simulink model "QDrone_YOLO_Integrated_Camera_Commander"  (R2021b)
settings: Solver=ode1  StartTime=0.0  StopTime=inf  FixedStep=0.001  RelTol=1e-3  EnableMultiTasking=on
InitFcn:
  | set_param(gcs, 'ZoomFactor','FitSystem')
model workspace (MAT data in the model file):
  target_system = 1
undefined symbols (not defined in the file): gcbh, HIL, JPEG, qc_get_step_size, video_display_show
libraries: quarc_library x53, simulink x23, simulink_extras x5
(part 2 of 3)

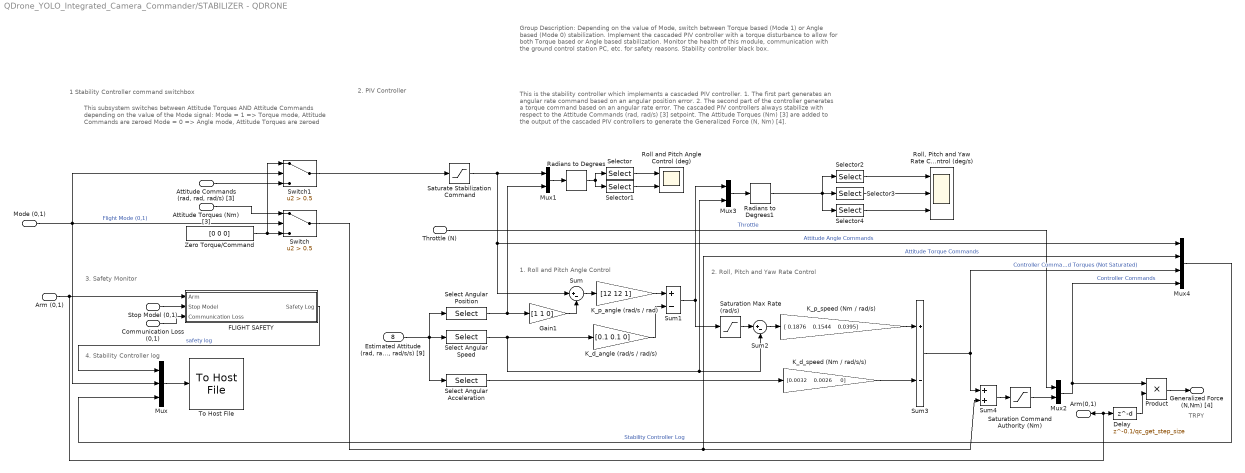
== system QDrone_YOLO_Integrated_Camera_Commander/STABILIZER - QDRONE  ==
  note: 2. PIV Controller
  note: 4. Stability Controller log
  note: 1 Stability Controller command switchbox
  note: Group Description:
      |
      | Depending on the value of Mode, switch between Torque based (Mode 1) or Angle based (Mode 0) stabilization.
      | Implement the cascaded PIV controller with a torque disturbance to allow for both Torque based or Angle based stabilization.
      | Monitor the health of this module, communication with the ground control station PC, etc. for safety reasons.
      | Stability controller black box.
  note: TRPY
  note: 2. Roll, Pitch and Yaw Rate Control
  note: 1. Roll and Pitch Angle Control
  note: This is the stability controller which implements a cascaded PIV controller.
      | 1. The first part generates an angular rate command based on an angular position error.
      | 2. The second part of the controller generates a torque command based on an angular rate error.
      |
      | The cascaded PIV controllers always stabilize with respect to the Attitude Commands (rad, rad/s) [3] setpoint. The Attitude Torques (Nm) [3] are added to the output of the cascaded PIV controllers to generate the Generalized Force (N, Nm) [4].
  note: This subsystem switches between Attitude Torques AND Attitude Commands depending on
      | the value of the Mode signal:
      | Mode = 1	=> 		Torque mode, Attitude Commands are zeroed
      | Mode = 0	=> 		Angle mode, Attitude Torques are zeroed
  note: 3. Safety Monitor
  Mode (0,1) : Inport
  Stop Model (0,1) : Inport  Port=2
  Throttle (N) : Inport  Port=3
  Attitude Torques (Nm) [3] : Inport  Port=4
  "Attitude Commands (rad, rad, rad/s) [3]" : Inport  Port=5
  Communication Loss (0,1) : Inport  Port=6
  Arm (0,1) : Inport  Port=7
  "Estimated Attitude (rad, rad/s, rad/s/s) [9]" : Inport  Port=8
  Delay : Delay  DelayLength=0.1/qc_get_step_size
  FLIGHT SAFETY : Subsystem
  Gain1 : Gain  Gain=[1 1 0]
  K_d_angle (rad/s / rad/s) : Gain  Gain=[0.1 0.1 0]
  K_d_speed (Nm / rad/s/s) : Gain  Gain="[0.0032    0.0026     0]"
  K_p_angle (rad/s / rad) : Gain  Gain=[12 12 1]
  K_p_speed (Nm / rad/s) : Gain  Gain="[ 0.1876    0.1544    0.0395]"
  Mux : Mux  Inputs=3
  Mux1 : Mux  Inputs=2
  Mux2 : Mux  Inputs=2
  Mux3 : Mux  Inputs=2
  Mux4 : Mux
  Product : Product
  Radians to Degrees : simulink_extras/Transformations/Radians to Degrees
  Radians to Degrees1 : simulink_extras/Transformations/Radians to Degrees
  Roll and Pitch Angle Control (deg) : Scope  NumInputPorts=2
  "Roll, Pitch and Yaw Rate Control (deg/s)" : Scope  NumInputPorts=3
  Saturate Stabilization Command : Saturate  UpperLimit=[pi/4 pi/4 10*pi/18]  LowerLimit=[-pi/4 -pi/4 -10*pi/18]
  Saturation Command Authority (Nm) : Saturate  UpperLimit=[1.0915 0.8984 0.0984]  LowerLimit=-[1.0915 0.8984 0.0984]
  Saturation Max Rate (rad/s) : Saturate  UpperLimit=10*pi/3*[1 1 1]  LowerLimit=-10*pi/3*[1 1 1]
  Select Angular Acceleration : Selector  InputPortWidth=9  IndexOptions=Index vector (dialog)  Indices=[7:9]  OutputSizes=1
  Select Angular Speed : Selector  InputPortWidth=9  IndexOptions=Index vector (dialog)  Indices=[4:6]  OutputSizes=1
  Select Angular Position : Selector  InputPortWidth=9  IndexOptions=Index vector (dialog)  Indices=[1:3]  OutputSizes=1
  Selector : Selector  InputPortWidth=6  IndexOptions=Index vector (dialog)  Indices=[1 4]  OutputSizes=1
  Selector1 : Selector  InputPortWidth=6  IndexOptions=Index vector (dialog)  Indices=[2 5]  OutputSizes=1
  Selector2 : Selector  InputPortWidth=6  IndexOptions=Index vector (dialog)  Indices=[1 4]  OutputSizes=1
  Selector3 : Selector  InputPortWidth=6  IndexOptions=Index vector (dialog)  Indices=[2 5]  OutputSizes=1
  Selector4 : Selector  InputPortWidth=6  IndexOptions=Index vector (dialog)  Indices=[3 6]  OutputSizes=1
  Sum : Sum  Inputs=|+-
  Sum1 : Sum  Inputs=+-
  Sum2 : Sum  Inputs=|+-
  Sum3 : Sum  Inputs=+-
  Sum4 : Sum
  Switch : Switch  Criteria=u2 > Threshold  Threshold=0.5
  Switch1 : Switch  Criteria=u2 > Threshold  Threshold=0.5
  To Host File : quarc_library/Sinks/To Host/To Host File  file_name=saved_data/%m/Stabilizer_%{date}_%{time}.mat  variable_name=stabilizer_data  decimation=1  sample_time=-1  file_format=MAT-file v.5  options=No header or footer  append=off  final_file_name=saved_data/QDrone_YOLO_Integrated_Camera_Commander/Stabilizer_19-Aug-2026_13-55-19.mat  bitrate=2000000
      settings: SourceProductName=The database C:\Users\user\AppData\Roaming\MathWorks\MATLAB\R2017a\slblocks_master.db is locked, or a table in the database is locked. (database is locked)
  Zero Torque/Command : Constant  Value=[0 0 0]
  Generalized Force (N,Nm) [4] : Outport  VectorParamsAs1DForOutWhenUnconnected=off
  Arm(0,1) : Outport  Port=2  VectorParamsAs1DForOutWhenUnconnected=off
  wires:
  Product/1 -> Generalized Force (N,Nm) [4]/1
  Stop Model (0,1)/1 -> FLIGHT SAFETY/2(Stop Model)
  Communication Loss (0,1)/1 -> FLIGHT SAFETY/3(Communication Loss)
  Mux/1 -> To Host File/1
  Mux4/1 -> Mux/3  "Stability Controller Log"
  Mode (0,1)/1 -> Switch/2, Switch1/2, Mux/2  "Flight Mode (0,1)"
  FLIGHT SAFETY/1(Safety Log) -> Mux/1  "safety log"
  K_p_speed (Nm / rad/s)/1 -> Sum3/1
  Sum/1 -> K_p_angle (rad/s / rad)/1
  K_d_speed (Nm / rad/s/s)/1 -> Sum3/2
  Arm (0,1)/1 -> Arm(0,1)/1, Delay/1, FLIGHT SAFETY/1(Arm)
  Mux3/1 -> Radians to Degrees1/1
  Sum1/1 -> Saturation Max Rate (rad/s)/1, Mux3/1
  Saturate Stabilization Command/1 -> Mux1/1, Sum/1, Mux4/1  "Attitude Angle Commands"
  Mux2/1 -> Mux4/4, Product/1  "Controller Commands"
  Select Angular Position/1 -> Mux1/2, Gain1/1
  Sum2/1 -> K_p_speed (Nm / rad/s)/1
  Throttle (N)/1 -> Mux2/1  "Throttle"
  Selector1/1 -> Roll and Pitch Angle Control (deg)/2
  Switch/1 -> Mux4/2, Sum4/2  "Attitude Torque Commands"
  Radians to Degrees1/1 -> Selector2/1, Selector4/1, Selector3/1
  "Estimated Attitude (rad, rad/s, rad/s/s) [9]"/1 -> Select Angular Position/1, Select Angular Acceleration/1, Select Angular Speed/1
  Mux1/1 -> Radians to Degrees/1
  Selector3/1 -> "Roll, Pitch and Yaw Rate Control (deg/s)"/2
  Sum4/1 -> Saturation Command Authority (Nm)/1
  Sum3/1 -> Mux4/3, Sum4/1  "Controller Command Torques (Not Saturated)"
  Saturation Command Authority (Nm)/1 -> Mux2/2
  Gain1/1 -> Sum/2
  Select Angular Acceleration/1 -> K_d_speed (Nm / rad/s/s)/1
  Switch1/1 -> Saturate Stabilization Command/1
  Saturation Max Rate (rad/s)/1 -> Sum2/1
  Selector4/1 -> "Roll, Pitch and Yaw Rate Control (deg/s)"/3
  K_p_angle (rad/s / rad)/1 -> Sum1/1
  Select Angular Speed/1 -> Sum2/2, Mux3/2, K_d_angle (rad/s / rad/s)/1
  Selector/1 -> Roll and Pitch Angle Control (deg)/1
  Selector2/1 -> "Roll, Pitch and Yaw Rate Control (deg/s)"/1
  K_d_angle (rad/s / rad/s)/1 -> Sum1/2
  Radians to Degrees/1 -> Selector/1, Selector1/1
  "Attitude Commands (rad, rad, rad/s) [3]"/1 -> Switch1/3
  Attitude Torques (Nm) [3]/1 -> Switch/1
  Zero Torque/Command/1 -> Switch1/1, Switch/3
  Delay/1 -> Product/2

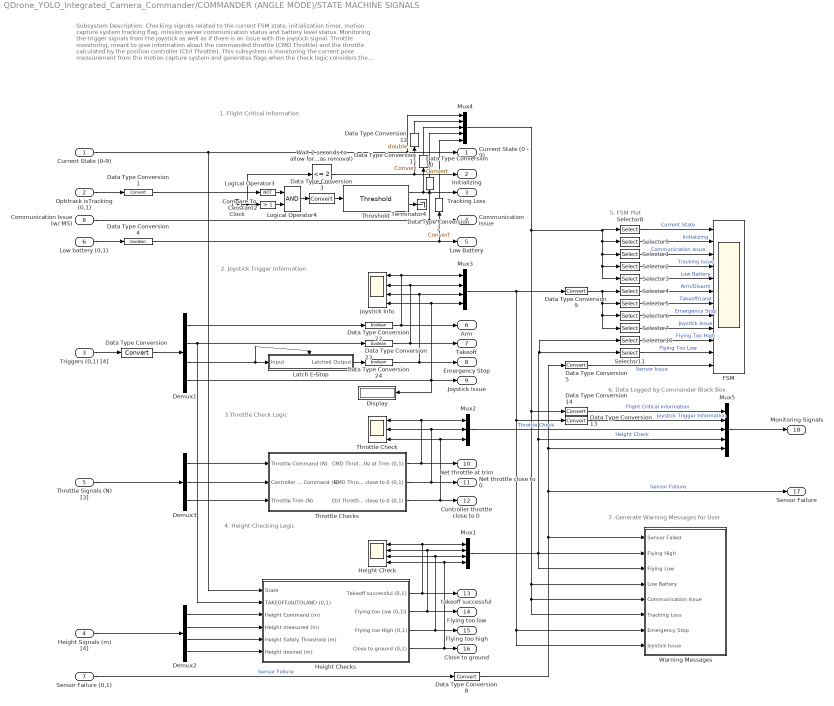
== system QDrone_YOLO_Integrated_Camera_Commander/COMMANDER (ANGLE MODE)/STATE MACHINE SIGNALS ==
  note: Subsystem Description:
      | Checking signals related to the current FSM state, initialization timer, motion capture system tracking flag, mission server communication status and battery level status.
      | Monitoring the trigger signals from the joystick as well as if there is an issue with the joystick signal.
      | Throttle monitoring, meant to give information about the commanded throttle (CMD Throttle) and the throttle calculated by the position controller (Ctrl Throttle).
      | This subsystem is monitoring the current pose measurement from the motion capture system and generates flags when the check logic considers the QDrone flying to close to ground, too high or too low as well as generate a successful take off flag.
      | A subset of the FSM monitoring signals are shown using this scope. These signals are what Quanser considers importnat for flight.
      | FSM signals sent to the blackbox for post flight monitoring.
      | Error message generation based on flags generated by the FSM signal checks.
  note: 7. Generate Warning Messages for User
  note: 5. FSM Plot
  note: 6. Data Logged by Commander Black Box
  note: 1. Flight Critical Information
  note: 2. Joystick Trigger Information
  note: 3.Throttle Check Logic
  note: 4. Height Checking Logic
  Current State (0-9) : Inport
  "Optitrack isTracking (0,1)  " : Inport  Port=2
  Triggers (0,1) [4] : Inport  Port=3
  Height Signals (m) [4] : Inport  Port=4
  Throttle Signals (N) [3] : Inport  Port=5
  Low battery (0,1) : Inport  Port=6
  Sensor Failure (0,1) : Inport  Port=7
  Communication Issue (w/ MS) : Inport  Port=8
  Clock : Clock
  Compare To Constant2 : simulink/Logic and Bit Operations/Compare To Constant  relop=>  const=1  OutDataTypeStr=boolean
  Data Type Conversion{,1..3,5,8..11,13..14} (11 alike) : DataTypeConversion
  Data Type Conversion12 : DataTypeConversion  OutDataTypeStr=double
  Data Type Conversion{4,22..24} (4 alike) : DataTypeConversion  OutDataTypeStr=boolean
  Demux1 : Demux  Outputs=[1 1 1 1]
  Demux2 : Demux
  Demux3 : Demux  Outputs=3
  Display : Display
  FSM : Scope  NumInputPorts=12
  "Height Check " : Scope  NumInputPorts=4
  Height Checks : Subsystem
  Joystick Info : Scope  NumInputPorts=4
  Latch E-Stop : Subsystem  TreatAsAtomicUnit=on
  Logical Operator3 : Logic  Operator=NOT  AllPortsSameDT=off  OutDataTypeStr=boolean
  Logical Operator4 : Logic  AllPortsSameDT=off  OutDataTypeStr=boolean
  Mux1 : Mux  Inputs=[1 1 1 1]
  Mux2 : Mux  Inputs=[1 1 1]
  Mux3 : Mux  Inputs=[1 1 1 1]
  Mux4 : Mux  Inputs=[1 1 1 1 1]
  Mux5 : Mux  Inputs=[5 4 3 4 1]
  Selector1 : Selector  InputPortWidth=5  IndexOptions=Index vector (dialog)  Indices=4  OutputSizes=1
  Selector10 : Selector  InputPortWidth=4  IndexOptions=Index vector (dialog)  Indices=3  OutputSizes=1
  Selector11 : Selector  InputPortWidth=4  IndexOptions=Index vector (dialog)  Indices=2  OutputSizes=1
  Selector2 : Selector  InputPortWidth=5  IndexOptions=Index vector (dialog)  Indices=3  OutputSizes=1
  Selector3 : Selector  InputPortWidth=5  IndexOptions=Index vector (dialog)  Indices=5  OutputSizes=1
  Selector4 : Selector  InputPortWidth=4  IndexOptions=Index vector (dialog)  Indices=1  OutputSizes=1
  Selector5 : Selector  InputPortWidth=4  IndexOptions=Index vector (dialog)  Indices=2  OutputSizes=1
  Selector6 : Selector  InputPortWidth=4  IndexOptions=Index vector (dialog)  Indices=3  OutputSizes=1
  Selector7 : Selector  InputPortWidth=4  IndexOptions=Index vector (dialog)  Indices=4  OutputSizes=1
  Selector8 : Selector  InputPortWidth=5  IndexOptions=Index vector (dialog)  Indices=1  OutputSizes=1
  Selector9 : Selector  InputPortWidth=5  IndexOptions=Index vector (dialog)  Indices=2  OutputSizes=1
  Terminator4 : Terminator
  Threshold : quarc_library/Discontinuities/Threshold  operator=>=  param_src=Specify via dialog  threshold=0.5  duration=0.2
      settings: SourceProductName=QUARC Targets
  Throttle Check : Scope  NumInputPorts=3
  Throttle Checks : Subsystem
  "Wait 2 seconds to allow for initialization (e.g., bias removal)" : simulink/Logic and Bit Operations/Compare To Constant  relop=<=  const=2  OutDataTypeStr=boolean
  Warning Messages : Subsystem
  "Current State (0 - 9)  " : Outport  VectorParamsAs1DForOutWhenUnconnected=off
  Initializing : Outport  Port=2  VectorParamsAs1DForOutWhenUnconnected=off
  Tracking Loss : Outport  Port=3  VectorParamsAs1DForOutWhenUnconnected=off
  Communication Issue : Outport  Port=4  VectorParamsAs1DForOutWhenUnconnected=off
  Low Battery : Outport  Port=5  VectorParamsAs1DForOutWhenUnconnected=off
  Arm : Outport  Port=6  VectorParamsAs1DForOutWhenUnconnected=off
  Takeoff : Outport  Port=7  VectorParamsAs1DForOutWhenUnconnected=off
  Emergency Stop : Outport  Port=8  VectorParamsAs1DForOutWhenUnconnected=off
  "Joystick Issue " : Outport  Port=9  VectorParamsAs1DForOutWhenUnconnected=off
  Net throttle at trim : Outport  Port=10  VectorParamsAs1DForOutWhenUnconnected=off
  Net throttle close to 0 : Outport  Port=11  VectorParamsAs1DForOutWhenUnconnected=off
  Controller throttle close to 0 : Outport  Port=12  VectorParamsAs1DForOutWhenUnconnected=off
  takeoff successful : Outport  Port=13  VectorParamsAs1DForOutWhenUnconnected=off
  Flying too low : Outport  Port=14  VectorParamsAs1DForOutWhenUnconnected=off
  Flying too high : Outport  Port=15  VectorParamsAs1DForOutWhenUnconnected=off
  Close to ground : Outport  Port=16  VectorParamsAs1DForOutWhenUnconnected=off
  "  Sensor Failure" : Outport  Port=17  VectorParamsAs1DForOutWhenUnconnected=off
  Monitoring Signals : Outport  Port=18  VectorParamsAs1DForOutWhenUnconnected=off
  wires:
  Triggers (0,1) [4]/1 -> Data Type Conversion/1
  Demux2/1 -> Height Checks/3(Height Command (m))
  Demux3/1 -> Throttle Checks/1(Throttle Command (N))
  Height Signals (m) [4]/1 -> Demux2/1
  Demux2/4 -> Height Checks/6(Height desired (m))
  Throttle Signals (N) [3]/1 -> Demux3/1
  Demux1/1 -> Data Type Conversion22/1
  Throttle Checks/2(CMD Throttle close to 0 (0,1)) -> Mux2/2, Throttle Check/2, Net throttle close to 0/1
  Height Checks/1(Takeoff successful (0,1)) -> takeoff successful/1, "Height Check "/1, Mux1/1
  Demux2/3 -> Height Checks/5(Height Safety Threshold (m))
  Demux1/2 -> Data Type Conversion23/1, Height Checks/2(TAKEOFF/AUTOLAND (0,1))
  Demux2/2 -> Height Checks/4(Height measured (m))
  Demux3/2 -> Throttle Checks/2(Controller Throttle Command (N))
  Demux3/3 -> Throttle Checks/3(Throttle Trim (N))
  Throttle Checks/1(CMD Throttle at Trim (0,1)) -> Net throttle at trim/1, Mux2/1, Throttle Check/1
  Height Checks/3(Flying too High (0,1)) -> Mux1/3, "Height Check "/3, Flying too high/1
  Height Checks/4(Close to ground (0,1)) -> "Height Check "/4, Mux1/4, Close to ground/1
  Data Type Conversion/1 -> Demux1/1
  Low battery (0,1)/1 -> Data Type Conversion4/1
  Height Checks/2(Flying too Low (0,1l)) -> Flying too low/1, Mux1/2, "Height Check "/2
  Sensor Failure (0,1)/1 -> Data Type Conversion8/1  "Sensor Failure"
  Data Type Conversion1/1 -> Logical Operator3/1
  Data Type Conversion3/1 -> Threshold/1
  Compare To Constant2/1 -> Logical Operator4/2
  Clock/1 -> "Wait 2 seconds to allow for initialization (e.g., bias removal)"/1, Compare To Constant2/1
  Logical Operator4/1 -> Data Type Conversion3/1
  Threshold/2 -> Terminator4/1
  Logical Operator3/1 -> Logical Operator4/1
  "Optitrack isTracking (0,1)  "/1 -> Data Type Conversion1/1
  Latch E-Stop/1(Latched Output) -> Data Type Conversion24/1
  Demux1/3 -> Latch E-Stop/1(Input), Latch E-Stop/Trigger
  Selector9/1 -> FSM/2  "Initializing"
  Selector1/1 -> FSM/3  "Communication Issue"
  Selector2/1 -> FSM/4  "Tracking Issue"
  Selector3/1 -> FSM/5  "Low Battery"
  Selector4/1 -> FSM/6  "Arm/Disarm"
  Selector5/1 -> FSM/7  "Takeoff/Land"
  Selector6/1 -> FSM/8  "Emergency Stop"
  Selector7/1 -> FSM/9  "Joystick Issue"
  Data Type Conversion5/1 -> FSM/12  "Sensor Issue"
  Selector10/1 -> FSM/10  "Flying Too High"
  Selector11/1 -> FSM/11  "Flying Too Low"
  Data Type Conversion24/1 -> Joystick Info/3, Mux3/3, Emergency Stop/1
  Data Type Conversion23/1 -> Joystick Info/2, Mux3/2, Takeoff/1
  Data Type Conversion22/1 -> Joystick Info/1, Mux3/1, Arm/1
  Data Type Conversion4/1 -> Low Battery/1, Data Type Conversion2/1
  Demux1/4 -> Display/1, Joystick Info/4, Mux3/4, "Joystick Issue "/1
  Communication Issue (w/ MS)/1 -> Communication Issue/1, Data Type Conversion10/1
  Threshold/1 -> Tracking Loss/1, Data Type Conversion11/1
  Mux5/1 -> Monitoring Signals/1
  Mux1/1 -> Warning Messages/3(Flying Low), Warning Messages/2(Flying High), Selector11/1, Selector10/1, Mux5/4  "Height Check"
  Mux2/1 -> Mux5/3  "Throttle Check"
  Mux3/1 -> Data Type Conversion9/1, Warning Messages/7("Emergency Stop "), Warning Messages/8(Joystick Issue), Data Type Conversion13/1
  Mux4/1 -> Warning Messages/4(Low Battery), Warning Messages/5(Communication Issue), Warning Messages/6(Tracking Loss), Data Type Conversion14/1, Selector3/1, Selector2/1, Selector1/1, Selector9/1, Selector8/1
  Throttle Checks/3(Ctrl Throttle close to 0 (0,1)) -> Mux2/3, Throttle Check/3, Controller throttle close to 0/1
  Data Type Conversion9/1 -> Selector4/1, Selector5/1, Selector7/1, Selector6/1
  Data Type Conversion8/1 -> "  Sensor Failure"/1, Data Type Conversion5/1, Mux5/5, Warning Messages/1(Sensor Failed)  "Sensor Failure"
  Current State (0-9)/1 -> Mux4/1, "Current State (0 - 9)  "/1, Height Checks/1(State)
  Selector8/1 -> FSM/1  "Current State"
  Data Type Conversion2/1 -> Mux4/5
  Data Type Conversion10/1 -> Mux4/4
  Data Type Conversion11/1 -> Mux4/3
  Data Type Conversion12/1 -> Mux4/2
  Data Type Conversion13/1 -> Mux5/2  "Joystick Trigger Information"
  Data Type Conversion14/1 -> Mux5/1  "Flight Critical information"
  "Wait 2 seconds to allow for initialization (e.g., bias removal)"/1 -> Data Type Conversion12/1, Initializing/1

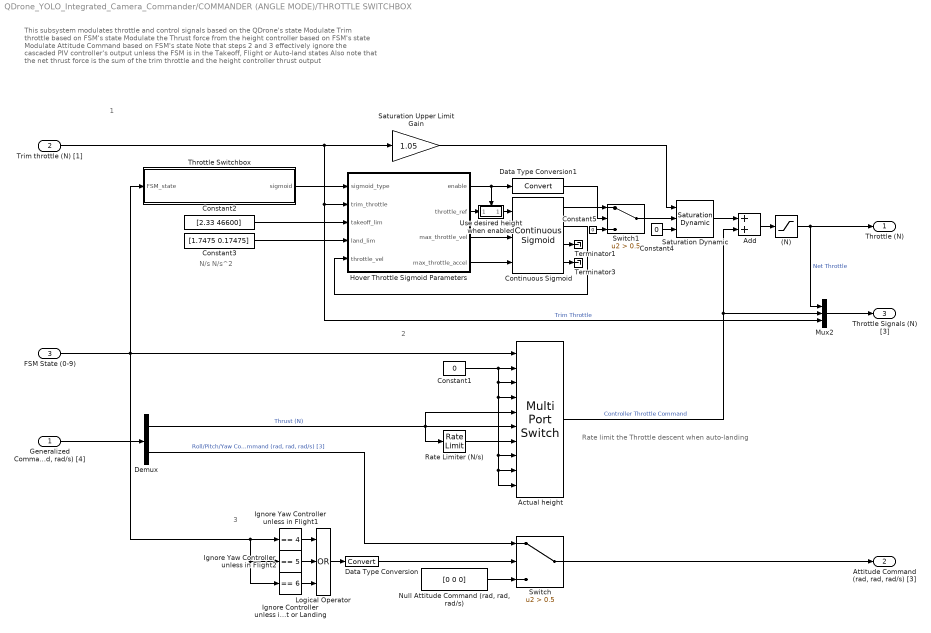
== system QDrone_YOLO_Integrated_Camera_Commander/COMMANDER (ANGLE MODE)/THROTTLE SWITCHBOX  ==
  note: 3
  note: 2
  note: 1
  note: Rate limit the Throttle descent when auto-landing
  note: This subsystem modulates throttle and control signals based on the QDrone's state
      | Modulate Trim throttle based on FSM's state
      | Modulate the Thrust force from the height controller based on FSM's state
      | Modulate Attitude Command based on FSM's state
      |
      | Note that steps 2 and 3 effectively ignore the cascaded PIV controller's output unless the FSM is in the Takeoff, Flight or Auto-land states
      | Also note that the net thrust force is the sum of the trim throttle and the height controller thrust output
  note: N/s N/s^2
  "Generalized Command (N, rad, rad, rad/s) [4]" : Inport
  Trim throttle (N) [1] : Inport  Port=2
  FSM State (0-9) : Inport  Port=3
  (N) : Saturate  UpperLimit=20.44  LowerLimit=0
  Actual height : MultiPortSwitch  Inputs=9
  Add : Sum
  Constant1 : Constant  Value=0
  Constant2 : Constant  Value=[2.33 46600]
  Constant3 : Constant  Value=[1.7475 0.17475]
  Constant4 : Constant  Value=0
  Constant5 : Constant  Value=0
  Continuous Sigmoid : quarc_library/Sources/Sigmoids/Continuous Sigmoid  params_source=External (input ports)  max_velocity=2  max_acceleration=10  initial_position=0  initial_velocity=0  hold_off=0.5  input_sample_time=-1  output_sample_time=qc_get_step_size
      settings: SourceProductName=QUARC Targets
  Data Type Conversion : DataTypeConversion
  Data Type Conversion1 : DataTypeConversion
  Demux : Demux  Outputs=[1 3]
  Hover Throttle Sigmoid Parameters : MATLAB Function  TreatAsAtomicUnit=on
  "Ignore Controller unless in Takeoff, Flight or Landing" : simulink/Logic and Bit Operations/Compare To Constant  relop===  const=6  OutDataTypeStr=boolean
  Ignore Yaw Controller unless in Flight1 : simulink/Logic and Bit Operations/Compare To Constant  relop===  const=4  OutDataTypeStr=boolean
  Ignore Yaw Controller unless in Flight2 : simulink/Logic and Bit Operations/Compare To Constant  relop===  const=5  OutDataTypeStr=boolean
  Logical Operator : Logic  Operator=OR  Inputs=3  AllPortsSameDT=off  OutDataTypeStr=boolean
  Mux2 : Mux  Inputs=3
  "Null Attitude Command (rad, rad, rad/s)" : Constant  Value=[0 0 0]
  Rate Limiter (N/s) : RateLimiter  RisingSlewLimit=100  FallingSlewLimit=-100  SampleTimeMode=inherited
  Saturation Dynamic : simulink/Discontinuities/Saturation Dynamic  OutMin=[]  OutMax=[]  OutDataTypeStr=Inherit: Same as second input  OutDataType=fixdt(1, 16)  OutScaling=2^-10  DoSatur=off
  Saturation Upper Limit Gain : Gain  Gain=1.05
  Switch : Switch  Criteria=u2 > Threshold  Threshold=0.5
  Switch1 : Switch  Criteria=u2 > Threshold  Threshold=0.5
  Terminator1 : Terminator
  Terminator3 : Terminator
  Throttle Switchbox : MATLAB Function  TreatAsAtomicUnit=on
  Use desired height when enabled : Subsystem  TreatAsAtomicUnit=on
  Throttle (N) : Outport  VectorParamsAs1DForOutWhenUnconnected=off
  "Attitude Command (rad, rad, rad/s) [3]" : Outport  Port=2  VectorParamsAs1DForOutWhenUnconnected=off
  Throttle Signals (N) [3] : Outport  Port=3  VectorParamsAs1DForOutWhenUnconnected=off
  wires:
  Actual height/1 -> Mux2/2, Add/2  "Controller Throttle Command"
  Add/1 -> (N)/1
  (N)/1 -> Mux2/1, Throttle (N)/1  "Net Throttle"
  "Generalized Command (N, rad, rad, rad/s) [4]"/1 -> Demux/1
  Mux2/1 -> Throttle Signals (N) [3]/1
  Ignore Yaw Controller unless in Flight2/1 -> Logical Operator/2
  Data Type Conversion/1 -> Switch/2
  "Null Attitude Command (rad, rad, rad/s)"/1 -> Switch/3
  Ignore Yaw Controller unless in Flight1/1 -> Logical Operator/1
  Demux/2 -> Switch/1  "Roll/Pitch/Yaw Command (rad, rad, rad/s) [3]"
  FSM State (0-9)/1 -> Actual height/1, "Ignore Controller unless in Takeoff, Flight or Landing"/1, Ignore Yaw Controller unless in Flight2/1, Ignore Yaw Controller unless in Flight1/1, Throttle Switchbox/1(FSM_state)
  "Ignore Controller unless in Takeoff, Flight or Landing"/1 -> Logical Operator/3
  Logical Operator/1 -> Data Type Conversion/1
  Demux/1 -> Actual height/6, Rate Limiter (N/s)/1, Actual height/5  "Thrust (N)"
  Continuous Sigmoid/2 -> Hover Throttle Sigmoid Parameters/5(throttle_vel)
  Constant4/1 -> Saturation Dynamic/3
  Saturation Dynamic/1 -> Add/1
  Constant3/1 -> Hover Throttle Sigmoid Parameters/4(land_lim)
  Switch1/1 -> Saturation Dynamic/2
  Trim throttle (N) [1]/1 -> Mux2/3, Hover Throttle Sigmoid Parameters/2(trim_throttle), Saturation Upper Limit Gain/1  "Trim Throttle"
  Throttle Switchbox/1(sigmoid) -> Hover Throttle Sigmoid Parameters/1(sigmoid_type)
  Saturation Upper Limit Gain/1 -> Saturation Dynamic/1
  Constant2/1 -> Hover Throttle Sigmoid Parameters/3(takeoff_lim)
  Hover Throttle Sigmoid Parameters/4(max_throttle_accel) -> Continuous Sigmoid/3
  Continuous Sigmoid/1 -> Switch1/1
  Continuous Sigmoid/4 -> Terminator3/1
  Hover Throttle Sigmoid Parameters/3(max_throttle_vel) -> Continuous Sigmoid/2
  Data Type Conversion1/1 -> Switch1/2
  Hover Throttle Sigmoid Parameters/1(enable) -> Data Type Conversion1/1, Use desired height when enabled/Enable
  Continuous Sigmoid/3 -> Terminator1/1
  Use desired height when enabled/1(Out1) -> Continuous Sigmoid/1
  Hover Throttle Sigmoid Parameters/2(throttle_ref) -> Use desired height when enabled/1(h_d (m) [1])
  Constant5/1 -> Switch1/3
  Switch/1 -> "Attitude Command (rad, rad, rad/s) [3]"/1
  Constant1/1 -> Actual height/8, Actual height/10, Actual height/9, Actual height/4, Actual height/3, Actual height/2
  Rate Limiter (N/s)/1 -> Actual height/7

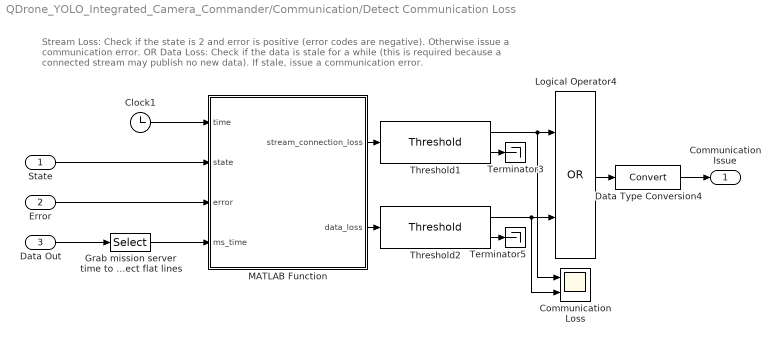
== system QDrone_YOLO_Integrated_Camera_Commander/Communication/Detect Communication Loss ==
  note: Stream Loss: Check if the state is 2 and error is positive (error codes are negative). Otherwise issue a communication error.
      | OR
      | Data Loss: Check if the data is stale for a while (this is required because a connected stream may publish no new data). If stale, issue a communication error.
  State : Inport
  Error : Inport  Port=2
  Data Out : Inport  Port=3
  Clock1 : Clock
  Communication Loss : Scope  NumInputPorts=2
  Data Type Conversion4 : DataTypeConversion
  Grab mission server time to detect flat lines : Selector  InputPortWidth=14  IndexOptions=Index vector (dialog)  Indices=[14]  OutputSizes=1
  Logical Operator4 : Logic  Operator=OR  AllPortsSameDT=off  OutDataTypeStr=boolean
  MATLAB Function : MATLAB Function  TreatAsAtomicUnit=on
  Terminator3 : Terminator
  Terminator5 : Terminator
  Threshold1 : quarc_library/Discontinuities/Threshold  operator=>=  param_src=Specify via dialog  threshold=0.5  duration=0.1
      settings: SourceProductName=QUARC Targets
  Threshold2 : quarc_library/Discontinuities/Threshold  operator=>=  param_src=Specify via dialog  threshold=0.5  duration=0.5
      settings: SourceProductName=QUARC Targets
  Communication Issue : Outport  VectorParamsAs1DForOutWhenUnconnected=off
  wires:
  Threshold2/1 -> Communication Loss/2, Logical Operator4/2
  Logical Operator4/1 -> Data Type Conversion4/1
  Threshold1/2 -> Terminator3/1
  MATLAB Function/2(data_loss) -> Threshold2/1
  MATLAB Function/1(stream_connection_loss) -> Threshold1/1
  Clock1/1 -> MATLAB Function/1(time)
  Threshold2/2 -> Terminator5/1
  Threshold1/1 -> Communication Loss/1, Logical Operator4/1
  Grab mission server time to detect flat lines/1 -> MATLAB Function/4(ms_time)
  Data Out/1 -> Grab mission server time to detect flat lines/1
  State/1 -> MATLAB Function/2(state)
  Error/1 -> MATLAB Function/3(error)
  Data Type Conversion4/1 -> Communication Issue/1

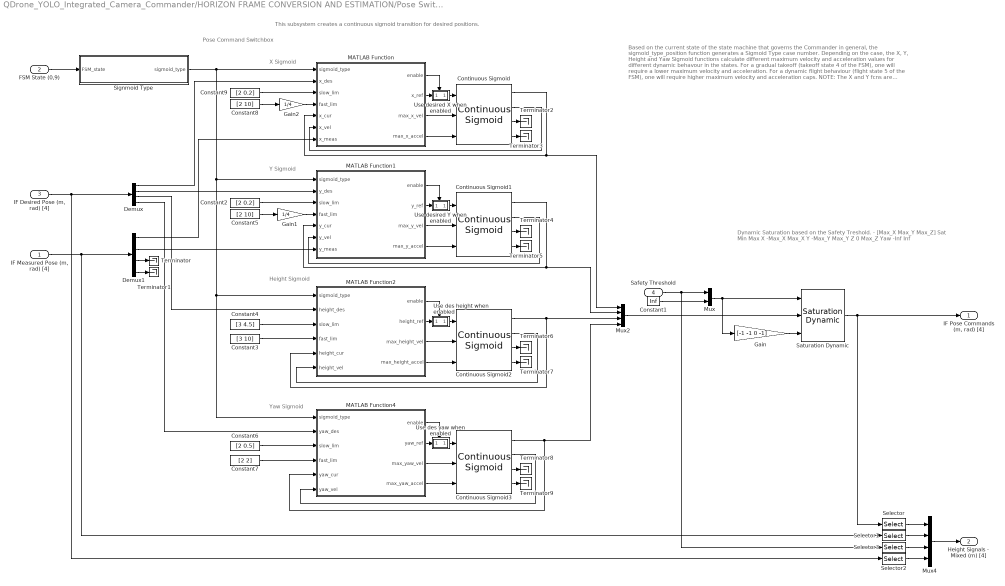
== system QDrone_YOLO_Integrated_Camera_Commander/HORIZON FRAME CONVERSION AND ESTIMATION/Pose Switchbox ==
  note: Dynamic Saturation based on the Safety Treshold. - [Max_X Max_Y Max_Z]
      |
      | Sat Min Max
      | X -Max_X Max_X
      | Y -Max_Y Max_Y
      | Z 0 Max_Z
      | Yaw -Inf Inf
  note: Based on the current state of the state machine that governs the Commander in general,
      | the sigmoid_type_position function generates a Sigmoid Type case number. Depending on
      | the case, the X, Y, Height and Yaw Sigmoid functions calculate different maximum velocity
      | and acceleration values for different dynamic behavour in the states.
      |
      | For a gradual takeoff (takeoff state 4 of the FSM), one will require a lower maximum velocity
      | and acceleration. For a dynamic flight behaviour (flight state 5 of the FSM), one will require
      | higher maximum velocity and acceleration caps.
      |
      | NOTE: The X and Y fcns are logically identical due to the generally symmetric X and Y behaviour.
      | The Z and Yaw fcns are different.
  note: This subsystem creates a continuous sigmoid transition for desired positions.
  note: Height Sigmoid
  note: Pose Command Switchbox
  note: X Sigmoid
  note: Yaw Sigmoid
  note: Y Sigmoid
  "IF Measured Pose (m, rad) [4]" : Inport
  FSM State (0,9) : Inport  Port=2
  "IF Desired Pose (m, rad) [4]" : Inport  Port=3
  Safety Threshold : Inport  Port=4
  Constant1 : Constant  Value=Inf
  Constant2 : Constant  Value=[2 0.2]
  Constant3 : Constant  Value=[3 10]
  Constant4 : Constant  Value=[3 4.5]
  Constant5 : Constant  Value=[2 10]
  Constant6 : Constant  Value=[2 0.5]
  Constant7 : Constant  Value=[2 2]
  Constant8 : Constant  Value=[2 10]
  Constant9 : Constant  Value=[2 0.2]
  Continuous Sigmoid{,1..3} (4 alike) : quarc_library/Sources/Sigmoids/Continuous Sigmoid  params_source=External (input ports)  max_velocity=2  max_acceleration=10  initial_position=0  initial_velocity=0  hold_off=0.5  input_sample_time=-1  output_sample_time=qc_get_step_size
      settings: SourceProductName=QUARC Targets
  Demux : Demux
  Demux1 : Demux
  Gain : Gain  Gain=[-1 -1 0 -1]
  Gain1 : Gain  Gain=1/4
  Gain2 : Gain  Gain=1/4
  MATLAB Function : MATLAB Function  TreatAsAtomicUnit=on
  MATLAB Function1 : MATLAB Function  TreatAsAtomicUnit=on
  MATLAB Function2 : MATLAB Function  TreatAsAtomicUnit=on
  MATLAB Function4 : MATLAB Function  TreatAsAtomicUnit=on
  Mux : Mux  Inputs=2
  Mux2 : Mux
  Mux4 : Mux
  Saturation Dynamic : simulink/Discontinuities/Saturation Dynamic  OutMin=[]  OutMax=[]  OutDataTypeStr=Inherit: Same as second input  OutDataType=fixdt(1, 16)  OutScaling=2^-10  DoSatur=off
  Selector : Selector  InputPortWidth=4  IndexOptions=Index vector (dialog)  Indices=[3]  OutputSizes=1
  Selector1 : Selector  InputPortWidth=4  IndexOptions=Index vector (dialog)  Indices=[3]  OutputSizes=1
  Selector2 : Selector  InputPortWidth=4  IndexOptions=Index vector (dialog)  Indices=[3]  OutputSizes=1
  Selector3 : Selector  InputPortWidth=3  IndexOptions=Index vector (dialog)  Indices=[3]  OutputSizes=1
  Signmoid Type : MATLAB Function  TreatAsAtomicUnit=on
  Terminator{,1..9} (10 alike) : Terminator
  Use des height when enabled : Subsystem  TreatAsAtomicUnit=on
  Use des yaw when enabled : Subsystem  TreatAsAtomicUnit=on
  Use desired X when enabled : Subsystem  TreatAsAtomicUnit=on
  Use desired Y when enabled : Subsystem  TreatAsAtomicUnit=on
  "IF Pose Commands (m, rad) [4]" : Outport  VectorParamsAs1DForOutWhenUnconnected=off
  Height Signals - Mixed (m) [4] : Outport  Port=2  VectorParamsAs1DForOutWhenUnconnected=off
  wires:
  Constant4/1 -> MATLAB Function2/3(slow_lim)
  Constant3/1 -> MATLAB Function2/4(fast_lim)
  Selector/1 -> Mux4/1
  Selector1/1 -> Mux4/2
  Selector2/1 -> Mux4/4
  Selector3/1 -> Mux4/3
  Safety Threshold/1 -> Mux/1, Selector3/1
  Mux/1 -> Saturation Dynamic/1, Gain/1
  Constant1/1 -> Mux/2
  Saturation Dynamic/1 -> "IF Pose Commands (m, rad) [4]"/1, Selector/1
  Mux2/1 -> Saturation Dynamic/2
  Mux4/1 -> Height Signals - Mixed (m) [4]/1
  Gain/1 -> Saturation Dynamic/3
  Demux/2 -> MATLAB Function1/2(y_des)
  Use desired Y when enabled/1(Out1) -> Continuous Sigmoid1/1
  Use desired X when enabled/1(Out1) -> Continuous Sigmoid/1
  MATLAB Function2/3(max_height_vel) -> Continuous Sigmoid2/2
  Continuous Sigmoid3/3 -> Terminator8/1
  Demux1/4 -> Terminator1/1
  MATLAB Function4/1(enable) -> Use des yaw when enabled/Enable
  Use des yaw when enabled/1(Out1) -> Continuous Sigmoid3/1
  Constant5/1 -> Gain1/1
  Continuous Sigmoid1/2 -> MATLAB Function1/6(y_vel)
  Constant2/1 -> MATLAB Function1/3(slow_lim)
  Constant6/1 -> MATLAB Function4/3(slow_lim)
  Demux1/1 -> MATLAB Function/7(x_meas)
  MATLAB Function1/2(y_ref) -> Use desired Y when enabled/1(h_d (m) [1])
  Demux/3 -> MATLAB Function2/2(height_des)
  Constant7/1 -> MATLAB Function4/4(fast_lim)
  Continuous Sigmoid1/4 -> Terminator5/1
  MATLAB Function1/1(enable) -> Use desired Y when enabled/Enable
  Continuous Sigmoid2/4 -> Terminator7/1
  Demux1/3 -> Terminator/1
  Signmoid Type/1(sigmoid_type) -> MATLAB Function/1(sigmoid_type), MATLAB Function1/1(sigmoid_type), MATLAB Function2/1(sigmoid_type), MATLAB Function4/1(sigmoid_type)
  MATLAB Function/3(max_x_vel) -> Continuous Sigmoid/2
  MATLAB Function2/1(enable) -> Use des height when enabled/Enable
  Constant9/1 -> MATLAB Function/3(slow_lim)
  Continuous Sigmoid2/2 -> MATLAB Function2/6(height_vel)
  Continuous Sigmoid1/1 -> MATLAB Function1/5(y_cur), Mux2/2
  MATLAB Function4/4(max_yaw_accel) -> Continuous Sigmoid3/3
  Demux/1 -> MATLAB Function/2(x_des)
  Constant8/1 -> Gain2/1
  MATLAB Function1/3(max_y_vel) -> Continuous Sigmoid1/2
  Continuous Sigmoid3/2 -> MATLAB Function4/6(yaw_vel)
  MATLAB Function2/2(height_ref) -> Use des height when enabled/1(h_d (m) [1])
  MATLAB Function/4(max_x_accel) -> Continuous Sigmoid/3
  Use des height when enabled/1(Out1) -> Continuous Sigmoid2/1
  Continuous Sigmoid2/3 -> Terminator6/1
  Demux/4 -> MATLAB Function4/2(yaw_des)
  MATLAB Function1/4(max_y_accel) -> Continuous Sigmoid1/3
  MATLAB Function/1(enable) -> Use desired X when enabled/Enable
  Continuous Sigmoid3/4 -> Terminator9/1
  MATLAB Function4/2(yaw_ref) -> Use des yaw when enabled/1(h_d (m) [1])
  FSM State (0,9)/1 -> Signmoid Type/1(FSM_state)
  MATLAB Function2/4(max_height_accel) -> Continuous Sigmoid2/3
  Continuous Sigmoid/4 -> Terminator3/1
  Continuous Sigmoid/3 -> Terminator2/1
  Continuous Sigmoid/1 -> MATLAB Function/5(x_cur), Mux2/1
  Continuous Sigmoid/2 -> MATLAB Function/6(x_vel)
  MATLAB Function/2(x_ref) -> Use desired X when enabled/1(h_d (m) [1])
  Continuous Sigmoid3/1 -> MATLAB Function4/5(yaw_cur), Mux2/4
  MATLAB Function4/3(max_yaw_vel) -> Continuous Sigmoid3/2
  Continuous Sigmoid2/1 -> MATLAB Function2/5(height_cur), Mux2/3
  Demux1/2 -> MATLAB Function1/7(y_meas)
  Continuous Sigmoid1/3 -> Terminator4/1
  "IF Measured Pose (m, rad) [4]"/1 -> Demux1/1, Selector1/1
  "IF Desired Pose (m, rad) [4]"/1 -> Demux/1, Selector2/1
  Gain1/1 -> MATLAB Function1/4(fast_lim)
  Gain2/1 -> MATLAB Function/4(fast_lim)

== system QDrone_YOLO_Integrated_Camera_Commander/PHYSICAL PLANT w// LINEAR THRUST/Check Battery level ==
  Battery level : Inport
  Compare To Constant : simulink/Logic and Bit Operations/Compare To Constant  relop=<=  const=10.5  OutDataTypeStr=boolean
  Compare To Constant1 : simulink/Logic and Bit Operations/Compare To Constant  relop=>  const=0.5  OutDataTypeStr=boolean
  Data Type Conversion : DataTypeConversion
  Data Type Conversion1 : DataTypeConversion
  Logical Operator : Logic  AllPortsSameDT=off  OutDataTypeStr=boolean
  Terminator : Terminator
  Threshold : quarc_library/Discontinuities/Threshold  operator=>=  param_src=Specify via dialog  threshold=0.5  duration=0.1
      settings: SourceProductName=The database C:\Users\user\AppData\Roaming\MathWorks\MATLAB\R2017a\slblocks_master.db is locked, or a table in the database is locked. (database is locked)
  Low Battery : Outport  VectorParamsAs1DForOutWhenUnconnected=off
  wires:
  Threshold/2 -> Terminator/1
  Battery level/1 -> Compare To Constant1/1, Compare To Constant/1
  Threshold/1 -> Logical Operator/2
  Logical Operator/1 -> Data Type Conversion1/1
  Compare To Constant1/1 -> Logical Operator/1
  Compare To Constant/1 -> Data Type Conversion/1
  Data Type Conversion/1 -> Threshold/1
  Data Type Conversion1/1 -> Low Battery/1

== system QDrone_YOLO_Integrated_Camera_Commander/PHYSICAL PLANT w// LINEAR THRUST/Red - Low Voltage Green - Armed Blue - Disarmed ==
  note: PCB LED 3
  note: PCB LED 2
  note: PCB LED 1
  note: PCB LED 5
  note: PCB LED 4
  note: Onboard LED
  Arm (0,1) : Inport
  Low Battery (0,1) : Inport  Port=2
  Blue : Constant  Value=[0 0 1]
  Green : Constant  Value=[0 1 0]
  MATLAB Function LED Color Assignment : MATLAB Function  TreatAsAtomicUnit=on
  Multiport Switch : MultiPortSwitch
  Mux : Mux  Inputs=[3 3 3 3 3 3]
  Red : Constant  Value=[1 0 0]
  LEDs (%) [18] : Outport  VectorParamsAs1DForOutWhenUnconnected=off
  wires:
  Multiport Switch/1 -> Mux/4, Mux/5, Mux/6, Mux/3, Mux/2, Mux/1
  Red/1 -> Multiport Switch/2
  Green/1 -> Multiport Switch/3
  Blue/1 -> Multiport Switch/4
  Arm (0,1)/1 -> MATLAB Function LED Color Assignment/1(arm)
  MATLAB Function LED Color Assignment/1(value) -> Multiport Switch/1
  Low Battery (0,1)/1 -> MATLAB Function LED Color Assignment/2(low_battery)
  Mux/1 -> LEDs (%) [18]/1

== system QDrone_YOLO_Integrated_Camera_Commander/PHYSICAL PLANT w// LINEAR THRUST/Sensor Failure Monitoring ==
  note: Check for no data condition (flat-line zero) from any of the onboard sensors
  Sensor Data [6] : Inport
  Data Type Conversion1 : DataTypeConversion
  Data Type Conversion2 : DataTypeConversion
  Data Type Conversion4 : DataTypeConversion
  Demux : Demux  Outputs=[3 3]
  Logical Operator : Logic  Operator=OR  Inputs=1  AllPortsSameDT=off  OutDataTypeStr=boolean
  Mux : Mux  Inputs=2
  Sensor Failure (Accelerometer) : Subsystem
  Sensor Failure (Gyroscope) : Subsystem
  Sensor Failure : Outport  VectorParamsAs1DForOutWhenUnconnected=off
  wires:
  Demux/2 -> Sensor Failure (Accelerometer)/1(Sensor Input)
  Sensor Failure (Gyroscope)/1(Sensor Fault) -> Data Type Conversion2/1
  Sensor Failure (Accelerometer)/1(Sensor Fault) -> Data Type Conversion1/1
  Mux/1 -> Logical Operator/1
  Data Type Conversion2/1 -> Mux/1
  Data Type Conversion1/1 -> Mux/2
  Sensor Data [6]/1 -> Demux/1
  Demux/1 -> Sensor Failure (Gyroscope)/1(Sensor Input)
  Logical Operator/1 -> Data Type Conversion4/1
  Data Type Conversion4/1 -> Sensor Failure/1

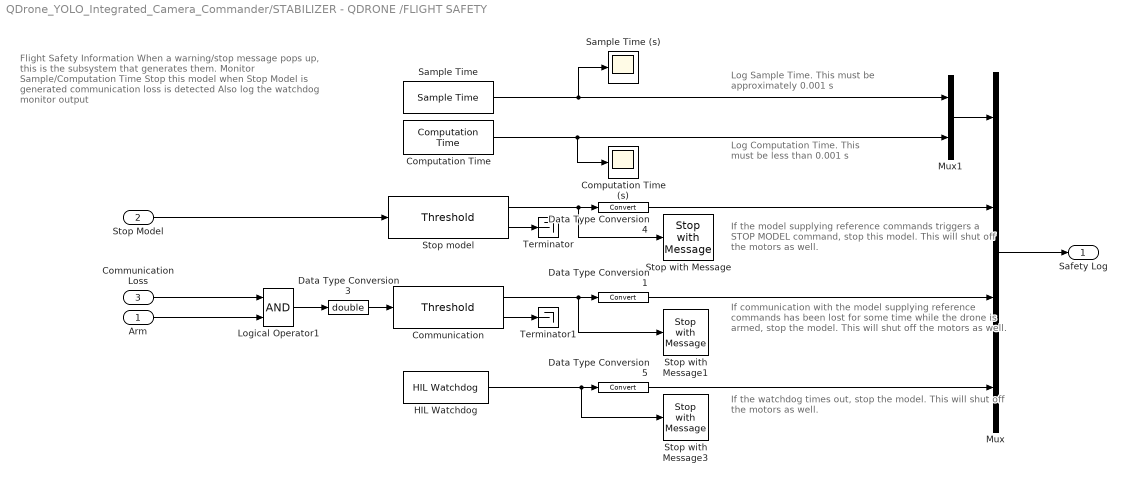
== system QDrone_YOLO_Integrated_Camera_Commander/STABILIZER - QDRONE /FLIGHT SAFETY ==
  note: Flight Safety Information
      |
      | When a warning/stop message pops up, this is the subsystem
      | that generates them.
      |
      | Monitor Sample/Computation Time
      | Stop this model
      | when Stop Model is generated
      | communication loss is detected
      | Also log the watchdog monitor output
  note: Log Sample Time. This must be approximately 0.001 s
  note: Log Computation Time. This must be less than 0.001 s
  note: If the model supplying reference commands triggers a STOP MODEL command, stop this model. This will shut off the motors as well.
  note: If communication with the model supplying reference commands has been lost for some time while the drone is armed, stop the model. This will shut off the motors as well.
  note: If the watchdog times out, stop the model. This will shut off the motors as well.
  Arm : Inport
  Stop Model : Inport  Port=2
  Communication Loss : Inport  Port=3
  Communication : quarc_library/Discontinuities/Threshold  operator=>=  param_src=Specify via dialog  threshold=0.5  duration=1
      settings: SourceProductName=The database C:\Users\user\AppData\Roaming\MathWorks\MATLAB\R2017a\slblocks_master.db is locked, or a table in the database is locked. (database is locked)
  Computation Time : quarc_library/Sources/Time/Computation Time  sample_time=qc_get_step_size  use_model=on  use_cpu_time=off
      settings: SourceProductName=The database C:\Users\user\AppData\Roaming\MathWorks\MATLAB\R2017a\slblocks_master.db is locked, or a table in the database is locked. (database is locked)
  Computation Time (s) : Scope
  Data Type Conversion1 : DataTypeConversion
  Data Type Conversion3 : DataTypeConversion  OutDataTypeStr=double
  Data Type Conversion4 : DataTypeConversion
  Data Type Conversion5 : DataTypeConversion
  HIL Watchdog : quarc_library/Data Acquisition/Generic/Watchdog/HIL Watchdog  object_name=HIL-1  timeout=0.1  sample_time=qc_get_step_size  active=off
      settings: AttributesFormatString=(%<object_name>)  SourceProductName=QUARC Targets
  Logical Operator1 : Logic  AllPortsSameDT=off  OutDataTypeStr=boolean
  Mux : Mux
  Mux1 : Mux  Inputs=2
  Sample Time : quarc_library/Sources/Time/Sample Time  Priority=-99  sample_time=qc_get_step_size
      settings: SourceProductName=The database C:\Users\user\AppData\Roaming\MathWorks\MATLAB\R2017a\slblocks_master.db is locked, or a table in the database is locked. (database is locked)
  Sample Time (s) : Scope
  Stop model : quarc_library/Discontinuities/Threshold  operator=>=  param_src=Specify via dialog  threshold=0.5  duration=0.1
      settings: SourceProductName=The database C:\Users\user\AppData\Roaming\MathWorks\MATLAB\R2017a\slblocks_master.db is locked, or a table in the database is locked. (database is locked)
  Stop with Message : quarc_library/Sinks/Error Handling/Stop with Message  message_type=Fixed error message  message_icon=Information  message=QDrone Stabilizer: Commander Terminated
      settings: SourceProductName=The database C:\Users\user\AppData\Roaming\MathWorks\MATLAB\R2017a\slblocks_master.db is locked, or a table in the database is locked. (database is locked)
  Stop with Message1 : quarc_library/Sinks/Error Handling/Stop with Message  message_type=Fixed error message  message_icon=Warning  message=QDrone Stabilizer: Communication with Commander lost
      settings: SourceProductName=The database C:\Users\user\AppData\Roaming\MathWorks\MATLAB\R2017a\slblocks_master.db is locked, or a table in the database is locked. (database is locked)
  Stop with Message3 : quarc_library/Sinks/Error Handling/Stop with Message  message_type=Fixed error message  message_icon=Information  message=QDrone Stabilizer: HIL Watchdog timer expired
      settings: SourceProductName=The database C:\Users\user\AppData\Roaming\MathWorks\MATLAB\R2017a\slblocks_master.db is locked, or a table in the database is locked. (database is locked)
  Terminator : Terminator
  Terminator1 : Terminator
  Safety Log : Outport  VectorParamsAs1DForOutWhenUnconnected=off
  wires:
  Mux/1 -> Safety Log/1
  Computation Time/1 -> Computation Time (s)/1, Mux1/2
  Sample Time/1 -> Sample Time (s)/1, Mux1/1
  Data Type Conversion4/1 -> Mux/2
  HIL Watchdog/1 -> Stop with Message3/1, Data Type Conversion5/1
  Stop model/2 -> Terminator/1
  Stop model/1 -> Data Type Conversion4/1, Stop with Message/1
  Stop Model/1 -> Stop model/1
  Communication/2 -> Terminator1/1
  Logical Operator1/1 -> Data Type Conversion3/1
  Data Type Conversion1/1 -> Mux/3
  Arm/1 -> Logical Operator1/2
  Communication/1 -> Data Type Conversion1/1, Stop with Message1/1
  Data Type Conversion3/1 -> Communication/1
  Communication Loss/1 -> Logical Operator1/1
  Mux1/1 -> Mux/1
  Data Type Conversion5/1 -> Mux/4

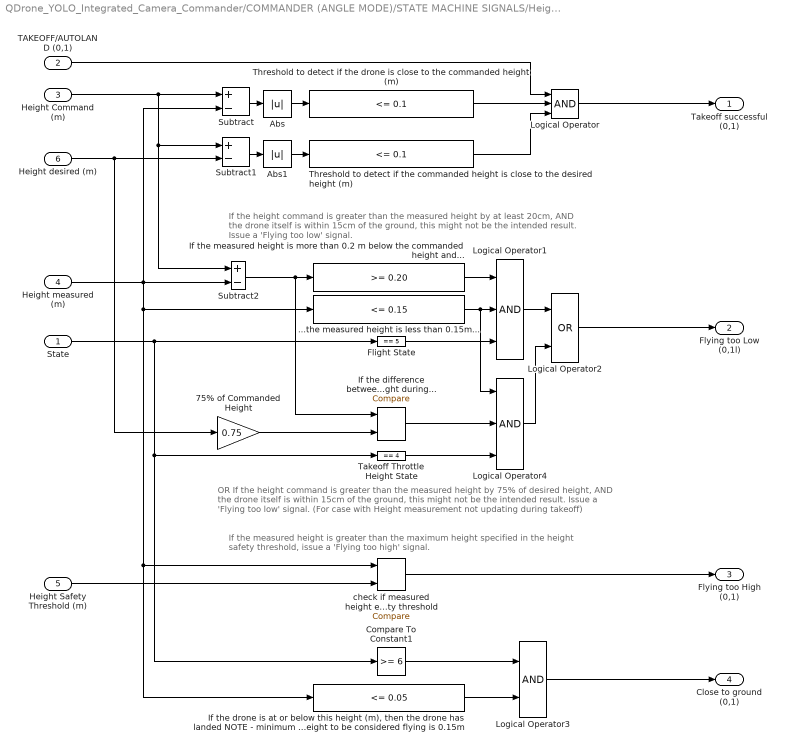
== system QDrone_YOLO_Integrated_Camera_Commander/COMMANDER (ANGLE MODE)/STATE MACHINE SIGNALS/Height Checks ==
  note: If the height command is greater than the measured height by at least 20cm, AND the drone itself is
      | within 15cm of the ground, this might not be the intended result. Issue a 'Flying too low' signal.
  note: If the measured height is greater than the maximum height specified in the height safety threshold,
      | issue a 'Flying too high' signal.
  note: OR If the height command is greater than the measured height by 75% of desired height, AND
      | the drone itself is within 15cm of the ground, this might not be the intended result. Issue a 'Flying too low' signal.
      | (For case with Height measurement not updating during takeoff)
  State : Inport
  TAKEOFF/AUTOLAND (0,1) : Inport  Port=2
  Height Command (m) : Inport  Port=3
  Height measured (m) : Inport  Port=4
  Height Safety Threshold (m) : Inport  Port=5
  Height desired (m) : Inport  Port=6
  ...the measured height is less than 0.15m... : simulink/Logic and Bit Operations/Compare To Constant  relop=<=  const=0.15  OutDataTypeStr=boolean
  75% of Commanded Height : Gain  Gain=0.75
  Abs : Abs
  Abs1 : Abs
  Compare To Constant1 : simulink/Logic and Bit Operations/Compare To Constant  relop=>=  const=6  OutDataTypeStr=boolean
  Flight State : simulink/Logic and Bit Operations/Compare To Constant  relop===  const=5  OutDataTypeStr=boolean
  If the difference between the measured and commanded height is greater than 75% of the commanded height during... : quarc_library/Logic Operations/Compare  operator=>=  output_data_type=boolean
      settings: SourceProductName=QUARC Targets
  "If the drone is at or below this height (m), then the drone has landed NOTE - minimum height to be considered flying is 0.15m   " : simulink/Logic and Bit Operations/Compare To Constant  relop=<=  const=0.05  OutDataTypeStr=boolean
  If the measured height is more than 0.2 m below the commanded height and... : simulink/Logic and Bit Operations/Compare To Constant  relop=>=  const=0.20  OutDataTypeStr=boolean
  Logical Operator : Logic  Inputs=3  AllPortsSameDT=off  OutDataTypeStr=boolean
  Logical Operator1 : Logic  Inputs=3  AllPortsSameDT=off  OutDataTypeStr=boolean
  Logical Operator2 : Logic  Operator=OR  AllPortsSameDT=off  OutDataTypeStr=boolean
  Logical Operator3 : Logic  AllPortsSameDT=off  OutDataTypeStr=boolean
  Logical Operator4 : Logic  Inputs=3  AllPortsSameDT=off  OutDataTypeStr=boolean
  Subtract : Sum  Inputs=+-
  Subtract1 : Sum  Inputs=+-
  Subtract2 : Sum  Inputs=+-
  Takeoff Throttle Height State : simulink/Logic and Bit Operations/Compare To Constant  relop===  const=4  OutDataTypeStr=boolean
  Threshold to detect if the commanded height is close to the desired height (m) : simulink/Logic and Bit Operations/Compare To Constant  relop=<=  const=0.1  OutDataTypeStr=boolean
  Threshold to detect if the drone is close to the commanded height (m) : simulink/Logic and Bit Operations/Compare To Constant  relop=<=  const=0.1  OutDataTypeStr=boolean
  check if measured height exceeds maximum height safety threshold : quarc_library/Logic Operations/Compare  operator=>=  output_data_type=boolean
      settings: SourceProductName=QUARC Targets
  Takeoff successful (0,1) : Outport  VectorParamsAs1DForOutWhenUnconnected=off
  Flying too Low (0,1l) : Outport  Port=2  VectorParamsAs1DForOutWhenUnconnected=off
  Flying too High (0,1) : Outport  Port=3  VectorParamsAs1DForOutWhenUnconnected=off
  Close to ground (0,1) : Outport  Port=4  VectorParamsAs1DForOutWhenUnconnected=off
  wires:
  Logical Operator/1 -> Takeoff successful (0,1)/1
  Logical Operator2/1 -> Flying too Low (0,1l)/1
  Subtract1/1 -> Abs1/1
  Threshold to detect if the commanded height is close to the desired height (m)/1 -> Logical Operator/3
  Abs/1 -> Threshold to detect if the drone is close to the commanded height (m)/1
  Threshold to detect if the drone is close to the commanded height (m)/1 -> Logical Operator/2
  Abs1/1 -> Threshold to detect if the commanded height is close to the desired height (m)/1
  Height desired (m)/1 -> 75% of Commanded Height/1, Subtract1/2
  TAKEOFF/AUTOLAND (0,1)/1 -> Logical Operator/1
  Subtract/1 -> Abs/1
  If the measured height is more than 0.2 m below the commanded height and.../1 -> Logical Operator1/1
  Logical Operator1/1 -> Logical Operator2/1
  Height Command (m)/1 -> Subtract1/1, Subtract2/1, Subtract/1
  ...the measured height is less than 0.15m.../1 -> Logical Operator4/1, Logical Operator1/2
  check if measured height exceeds maximum height safety threshold/1 -> Flying too High (0,1)/1
  Height Safety Threshold (m)/1 -> check if measured height exceeds maximum height safety threshold/2
  State/1 -> Flight State/1, Takeoff Throttle Height State/1, Compare To Constant1/1
  Logical Operator3/1 -> Close to ground (0,1)/1
  "If the drone is at or below this height (m), then the drone has landed NOTE - minimum height to be considered flying is 0.15m   "/1 -> Logical Operator3/2
  Compare To Constant1/1 -> Logical Operator3/1
  Height measured (m)/1 -> Subtract/2, ...the measured height is less than 0.15m.../1, "If the drone is at or below this height (m), then the drone has landed NOTE - minimum height to be considered flying is 0.15m   "/1, check if measured height exceeds maximum height safety threshold/1, Subtract2/2
  Logical Operator4/1 -> Logical Operator2/2
  Flight State/1 -> Logical Operator1/3
  Subtract2/1 -> If the difference between the measured and commanded height is greater than 75% of the commanded height during.../1, If the measured height is more than 0.2 m below the commanded height and.../1
  Takeoff Throttle Height State/1 -> Logical Operator4/3
  75% of Commanded Height/1 -> If the difference between the measured and commanded height is greater than 75% of the commanded height during.../2
  If the difference between the measured and commanded height is greater than 75% of the commanded height during.../1 -> Logical Operator4/2

== system QDrone_YOLO_Integrated_Camera_Commander/COMMANDER (ANGLE MODE)/STATE MACHINE SIGNALS/Latch E-Stop ==
  Input : Inport
  Trigger : TriggerPort  VariantControl=Variant
  Latched Output : Outport  InitialOutput=0  VectorParamsAs1DForOutWhenUnconnected=off
  wires:
  Input/1 -> Latched Output/1

== system QDrone_YOLO_Integrated_Camera_Commander/COMMANDER (ANGLE MODE)/STATE MACHINE SIGNALS/Throttle Checks ==
  Throttle Command (N) : Inport
  Controller Throttle Command (N) : Inport  Port=2
  Throttle Trim (N) : Inport  Port=3
  Abs : Abs
  Abs1 : Abs
  Subtract : Sum  Inputs=+-
  Threshold below which throttle can be assumed to be close to zero (N) (17.1% of Max Thrust) : simulink/Logic and Bit Operations/Compare To Constant  relop=<=  const=3.5  OutDataTypeStr=boolean
  Threshold to determine if the controller throttle is close to zero (N) (6.8% of Max Thrust) : simulink/Logic and Bit Operations/Compare To Constant  relop=<=  const=1.40  OutDataTypeStr=boolean
  Threshold to determine if throttle is close to the trim value (N) (3.4% of Max Thrust) : simulink/Logic and Bit Operations/Compare To Constant  relop=<=  const=0.7  OutDataTypeStr=boolean
  CMD Throttle at Trim (0,1) : Outport  VectorParamsAs1DForOutWhenUnconnected=off
  CMD Throttle close to 0 (0,1) : Outport  Port=2  VectorParamsAs1DForOutWhenUnconnected=off
  Ctrl Throttle close to 0 (0,1) : Outport  Port=3  VectorParamsAs1DForOutWhenUnconnected=off
  wires:
  Throttle Command (N)/1 -> Subtract/1, Threshold below which throttle can be assumed to be close to zero (N) (17.1% of Max Thrust)/1
  Throttle Trim (N)/1 -> Subtract/2
  Abs/1 -> Threshold to determine if throttle is close to the trim value (N) (3.4% of Max Thrust)/1
  Subtract/1 -> Abs/1
  Threshold to determine if throttle is close to the trim value (N) (3.4% of Max Thrust)/1 -> CMD Throttle at Trim (0,1)/1
  Threshold below which throttle can be assumed to be close to zero (N) (17.1% of Max Thrust)/1 -> CMD Throttle close to 0 (0,1)/1
  Abs1/1 -> Threshold to determine if the controller throttle is close to zero (N) (6.8% of Max Thrust)/1
  Controller Throttle Command (N)/1 -> Abs1/1
  Threshold to determine if the controller throttle is close to zero (N) (6.8% of Max Thrust)/1 -> Ctrl Throttle close to 0 (0,1)/1
